simulink model "s_b4a4x32kf_54"  (R2018a)
(part 2 of 274)

  acc_len/1(in_reg) -> Delay21/1(d)
  [gbe_rxvld] -> pipeline76/1(d)
  [gbe_rxdata] -> pipeline75/1(d)
  [gbe_rxeof] -> pipeline77/1(d)
  gbe_porttx/1(in_reg) -> Delay9/1(d)
  gbe_iptx/1(in_reg) -> Delay10/1(d)
  Delay9/1(q) -> [gbe_porttx]
  Delay10/1(q) -> [gbe_iptx]
  board_id/1(in_reg) -> Delay72/1(d)
  unpack_feng_hardcoded/1(pkt_start) -> Terminator28/1
  unpack_feng_hardcoded/2(data256) -> pipeline34/1(d)
  unpack_feng_hardcoded/3(valid256) -> pipeline46/1(d)
  unpack_feng_hardcoded/4(eof256) -> pipeline47/1(d)
  Delay72/1(q) -> [board_id]
  vacc_time_msw/3(in_msw) -> Delay19/1(d)
  vacc_time_msw/1(in_arm) -> Delay16/1(d)
  Concat10/1 -> [vacc_ld_time]
  vacc_time_msw/2(in_immediate) -> Delay18/1(d)
  vacc_time_lsw/1(in_lsw) -> Delay20/1(d)
  Delay16/1(q) -> [vacc_ld_arm]
  Delay18/1(q) -> [vacc_ld_immediate]
  Delay19/1(q) -> Concat10/1
  Delay20/1(q) -> Concat10/2
  Delay21/1(q) -> [acc_len]
  pipeline24/1(q) -> [gap_size3]
  pipeline23/1(q) -> [gap_size2]
  pipeline14/1(q) -> [gap_size1]
  pipeline10/1(q) -> [gap_size0]
  gapsize/1(in_gap_size) -> Register/1, Relational/2, Delay1/1
  Delay1/1 -> Relational/1
  Register/1 -> pipeline24/1(d), pipeline23/1(d), pipeline14/1(d), pipeline10/1(d)
  bf_config/1(in_data_id) -> pipeline26/1(d)
  bf_config/2(in_time_id) -> pipeline27/1(d)
  bf_weight/1(in_stream) -> pipeline29/1(d)
  bf_weight/2(in_antenna) -> pipeline30/1(d)
  pipeline26/1(q) -> [bf_data_id]
  pipeline27/1(q) -> [bf_time_id]
  pipeline29/1(q) -> [bf_stream]
  pipeline30/1(q) -> [bf_antenna]
  pipeline55/1(q) -> [bf_value_bw]
  pipeline33/1(q) -> edge_detect7/1(in)
  [bfout_valbw0] -> Delay27/1(d)
  [bfout_valbw1] -> Delay26/1(d)
  [bfout_valbw2] -> Delay28/1(d)
  [bfout_valbw3] -> Delay32/1(d)
  Delay27/1(q) -> bf_valout_bw0/1(out_bw0)
  Delay26/1(q) -> bf_valout_bw0/2(out_bw1)
  Delay32/1(q) -> bf_valout_bw1/2(out_bw3)
  Delay28/1(q) -> bf_valout_bw1/1(out_bw2)
  edge_detect7/1(out) -> [bf_valctrl_bw]
  pipeline59/1(q) -> [bf_tvgsel]
  bf_config/3(in_tvg_sel) -> pipeline59/1(d)
  pipeline60/1(q) -> [bf_snap_arm]
  pipeline61/1(q) -> [bf_snap_trig]
  bf_config/4(in_snap_arm) -> pipeline60/1(d)
  bf_config/5(in_snap_trig) -> pipeline61/1(d)
  pipeline43/1(q) -> [bf1_txport]
  pipeline44/1(q) -> [bf1_txen]
  pipeline35/1(q) -> [bf0_txport]
  pipeline36/1(q) -> [bf0_txen]
  pipeline51/1(q) -> [bf0_txip]
  pipeline52/1(q) -> [bf1_txip]
  pipeline73/1(q) -> Convert/1
  pipeline74/1(q) -> Convert1/1
  gbe0/1(led_up) -> [gbe_up]
  gbe0/2(led_rx) -> Terminator1/1
  gbe0/3(led_tx) -> Terminator6/1
  gbe0/4(tx_afull) -> Terminator8/1
  gbe0/5(tx_overflow) -> [gbe_tx_over]
  gbe0/6(rx_data) -> [gbe_rxdata]
  gbe0/8(rx_source_ip) -> [gbe_src_ip]
  gbe0/9(rx_source_port) -> [gbe_src_port]
  gbe0/10(rx_end_of_frame) -> [gbe_rxeof]
  gbe0/11(rx_bad_frame) -> [gbe_rx_bad]
  gbe0/12(rx_overrun) -> [gbe_rx_overrun]
  gbe0/14(rx_dest_port) -> [gbe_dest_port]
  gbe0/13(rx_dest_ip) -> [gbe_dest_ip]
  [gbe_rst] -> gbe0/1(rst)
  [gbe_txd] -> gbe0/2(tx_data)
  [gbe_txip] -> gbe0/4(tx_dest_ip)
  [gbe_txport] -> gbe0/5(tx_dest_port)
  [gbe_txeof] -> gbe0/6(tx_end_of_frame)
  Constant3/1 -> gbe0/7(rx_ack)
  Constant4/1 -> gbe0/8(rx_overrun_ack)
  [gbe_debug_rst] -> gbe0/9(debug_rst)
  unpack_feng_hardcoded/13(hdr5_0x1600_DIR) -> pipeline49/1(d)
  unpack_feng_hardcoded/9(hdr_heap_id) -> Terminator2/1
  unpack_feng_hardcoded/10(hdr_heap_size) -> Terminator3/1
  unpack_feng_hardcoded/11(hdr_heap_offset) -> pipeline48/1(d)
  unpack_feng_hardcoded/12(hdr_pkt_len) -> Terminator5/1
  unpack_feng_hardcoded/14(hdr6_0x4101_DIR) -> pipeline53/1(d)
  unpack_feng_hardcoded/16(hdr8_0x4300) -> Terminator31/1
  unpack_feng_hardcoded/15(hdr7_0x4103_DIR) -> pipeline56/1(d)
  pipeline77/1(q) -> unpack_feng_hardcoded/3(pkt_eof)
  pipeline76/1(q) -> unpack_feng_hardcoded/2(pkt_valid)
  pipeline75/1(q) -> unpack_feng_hardcoded/1(pkt_data)
  Concat8/1 -> gbe_mux_bus/1(di)
  [pack_txd1] -> Concat8/2
  [pack_txd0] -> Concat8/1
  Concat11/1 -> gbe_mux_bus/2(validi)
  Concat2/1 -> gbe_mux_bus/3(eofi)
  gbe_mux_bus/5(start) -> bus_expand1/1(bus_in), Delay6/1
  Concat3/1 -> gbe_mux_bus/4(drdy)
  Constant2/1 -> gbe_mux_bus/5(transmit)
  gbe_mux_bus/2(do) -> Delay7/1
  gbe_mux_bus/3(valido) -> Delay17/1
  gbe_mux_bus/4(eofo) -> Delay25/1
  gbe_mux_bus/6(flush) -> [flush]
  [bf0s_d0] -> Concat8/3
  [bf1s_d0] -> Concat8/4
  [pack_txvld0] -> Concat11/1
  [pack_txvld1] -> Concat11/2
  [bf0s_en0] -> Concat11/3
  [bf1s_en0] -> Concat11/4
  [bf0s_eof0] -> Concat2/3
  [bf1s_eof0] -> Concat2/4
  [pack_txeof0] -> Concat2/1
  [pack_txeof1] -> Concat2/2
  [bf0s_pkt_ready0] -> Concat3/3
  [bf1s_pkt_ready0] -> Concat3/4
  [pack_ready1] -> Concat3/2
  [pack_ready0] -> Concat3/1
  [bf0s_d1] -> Concat8/5
  [bf1s_d1] -> Concat8/6
  [bf0s_en1] -> Concat11/5
  [bf1s_en1] -> Concat11/6
  [bf0s_eof1] -> Concat2/5
  [bf1s_eof1] -> Concat2/6
  [bf0s_pkt_ready1] -> Concat3/5
  [bf1s_pkt_ready1] -> Concat3/6
  Delay7/1 -> [gbe_txd]
  Delay17/1 -> [gbe_txvld]
  Delay25/1 -> [gbe_txeof]
  [bf0_txport] -> Mux6/6, Mux6/4
  [bf1_txport] -> Mux6/5, Mux6/7
  [gbe_porttx] -> Mux6/3, Mux6/2
  Mux6/1 -> [gbe_txport]
  gbe_mux_bus/1(input) -> [gbe_ipsel]
  Delay6/1 -> [gbe_txstart]
  Mux5/1 -> [gbe_txip]
  [bf0_txport] -> Mux6/12, Mux6/10
  [bf1_txport] -> Mux6/13, Mux6/11
  [gbe_porttx] -> Mux6/9, Mux6/8
  bus_expand1/12(lsb_out1) -> [bf1_tx_pkt3]
  bus_expand1/1(msb_out12) -> [go0]
  bus_expand1/2(out11) -> [go1]
  bus_expand1/3(out10) -> [bf0_tx_pkt0]
  bus_expand1/4(out9) -> [bf1_tx_pkt0]
  bus_expand1/5(out8) -> [bf0_tx_pkt1]
  bus_expand1/6(out7) -> [bf1_tx_pkt1]
  bus_expand1/7(out6) -> [go2]
  bus_expand1/8(out5) -> [go3]
  bus_expand1/9(out4) -> [bf0_tx_pkt2]
  bus_expand1/10(out3) -> [bf1_tx_pkt2]
  bus_expand1/11(out2) -> [bf0_tx_pkt3]
  [gbe_iptx] -> Concat/1
  [gbe_iptx] -> Concat/2
  [bf0_txip] -> Concat/3
  [bf1_txip] -> Concat/4
  [bf0_txip] -> Concat/5
  [bf1_txip] -> Concat/6
  [gbe_iptx] -> Concat/7
  [gbe_iptx] -> Concat/8
  [bf0_txip] -> Concat/9
  [bf1_txip] -> Concat/10
  [bf0_txip] -> Concat/11
  [bf1_txip] -> Concat/12
  Concat/1 -> bus_addsub/1(a)
  [id2] -> Concat1/9
  [id3] -> Concat1/12
  [id1] -> Concat1/2
  [id0] -> Concat1/1
  [id1] -> Concat1/5
  [id0] -> Concat1/4
  [id3] -> Concat1/8
  [id1] -> Concat1/6
  [id3] -> Concat1/11
  [id2] -> Concat1/10
  [id0] -> Concat1/3
  [id2] -> Concat1/7
  Concat1/1 -> bus_addsub/2(b)
  bus_addsub/1(dout) -> bus_expand/1(bus_in)
  bus_expand/1(msb_out12) -> Mux5/2
  bus_expand/2(out11) -> Mux5/3
  bus_expand/3(out10) -> Mux5/4
  bus_expand/4(out9) -> Mux5/5
  bus_expand/5(out8) -> Mux5/6
  bus_expand/6(out7) -> Mux5/7
  bus_expand/7(out6) -> Mux5/8
  bus_expand/8(out5) -> Mux5/9
  bus_expand/9(out4) -> Mux5/10
  bus_expand/10(out3) -> Mux5/11
  bus_expand/11(out2) -> Mux5/12
  bus_expand/12(lsb_out1) -> Mux5/13
  [pack_txd2] -> Concat8/7
  [pack_txd3] -> Concat8/8
  [pack_txvld2] -> Concat11/7
  [pack_txvld3] -> Concat11/8
  [pack_txeof2] -> Concat2/7
  [pack_txeof3] -> Concat2/8
  [pack_ready2] -> Concat3/7
  [pack_ready3] -> Concat3/8
  [bf0s_d2] -> Concat8/9
  [bf1s_d2] -> Concat8/10
  [bf0s_d3] -> Concat8/11
  [bf1s_d3] -> Concat8/12
  [bf0s_en2] -> Concat11/9
  [bf1s_en2] -> Concat11/10
  [bf0s_en3] -> Concat11/11
  [bf1s_en3] -> Concat11/12
  [bf0s_eof2] -> Concat2/9
  [bf1s_eof2] -> Concat2/10
  [bf0s_eof3] -> Concat2/11
  [bf1s_eof3] -> Concat2/12
  [bf0s_pkt_ready2] -> Concat3/9
  [bf1s_pkt_ready2] -> Concat3/10
  [bf0s_pkt_ready3] -> Concat3/11
  [bf1s_pkt_ready3] -> Concat3/12
  Relational/1 -> Register/2
  [gbe_ipsel] -> Mux5/1
  [gbe_ipsel] -> Mux6/1
  [gbe_txvld] -> gbe0/3(tx_valid)
  gbe0/7(rx_valid) -> [gbe_rxvld]
  unpack_feng_hardcoded/5(magic_error) -> [spead_magic_err]
  unpack_feng_hardcoded/6(hdr_error) -> [spead_hdr_err]
  unpack_feng_hardcoded/7(pad_error) -> [spead_pad_err]
  unpack_feng_hardcoded/8(pkt_len_err) -> [spead_pkt_len_err]
  [spead_pkt_len_err] -> Subsystem2/5(in3)
  [spead_pad_err] -> Subsystem2/4(in2)
  Subsystem2/4(out3) -> spead_status0/4(out_pkt_len_err_cnt)
  Subsystem2/3(out2) -> spead_status0/3(out_pad_err_cnt)
  Subsystem2/2(out1) -> spead_status0/2(out_header_err_cnt)
  Subsystem2/1(out0) -> spead_status0/1(out_magic_err_cnt)
  [cnt_rst] -> Subsystem2/1(rst)
  [spead_magic_err] -> Subsystem2/2(in0)
  [spead_hdr_err] -> Subsystem2/3(in1)
  [gbe_rxvld] -> Delay48/1
  [gbe_rxdata] -> Slice5/1
  [gbe_rxeof] -> Delay49/1
  [gbe_dest_ip] -> Delay50/1
  [gbe_rx_overrun] -> Delay55/1
  [gbe_src_ip] -> Delay52/1
  [gbe_dest_port] -> Delay51/1
  [gbe_src_port] -> Delay53/1
  [gbe_rx_bad] -> Delay54/1
  [gbe_rxvld] -> Delay56/1
  [gbe_rxeof] -> Delay57/1
  [spead_pkt_len_err] -> Logical4/4
  [spead_pad_err] -> Logical4/3
  [spead_hdr_err] -> Logical4/2
  [spead_magic_err] -> Logical4/1
  Logical4/1 -> snap_gbe0_rx/12(stop)
  Delay47/1 -> snap_gbe0_rx/1(in_data)
  Delay48/1 -> snap_gbe0_rx/2(in_valid)
  Delay49/1 -> snap_gbe0_rx/3(in_eof)
  Delay50/1 -> snap_gbe0_rx/4(in_dest_ip)
  Delay51/1 -> snap_gbe0_rx/5(in_dest_port)
  Delay52/1 -> snap_gbe0_rx/6(in_src_ip)
  Delay53/1 -> snap_gbe0_rx/7(in_src_port)
  Delay54/1 -> snap_gbe0_rx/8(in_rx_bad)
  Delay55/1 -> snap_gbe0_rx/9(in_rx_over)
  Delay56/1 -> snap_gbe0_rx/10(we)
  Delay57/1 -> snap_gbe0_rx/11(trig)
  Delay58/1 -> snap_gbe0_rx/13(arm)
  Slice5/1 -> Delay47/1
  [gbe_ipsel] -> Delay81/1
  [gbe_txeof] -> snap_pack_mux/2(in_eof)
  Delay81/1 -> snap_pack_mux/1(in_input_select)
  [gbe_txvld] -> snap_pack_mux/52(we)
  [go3] -> snap_pack_mux/6(in_go3)
  [go2] -> snap_pack_mux/5(in_go2)
  [go1] -> snap_pack_mux/4(in_go1)
  [go0] -> snap_pack_mux/3(in_go0)
  [bf0_tx_pkt0] -> snap_pack_mux/7(in_bf0_tx_pkt0)
  [bf0_tx_pkt1] -> snap_pack_mux/8(in_bf0_tx_pkt1)
  [bf0_tx_pkt2] -> snap_pack_mux/9(in_bf0_tx_pkt2)
  [bf0_tx_pkt3] -> snap_pack_mux/10(in_bf0_tx_pkt3)
  [bf1_tx_pkt0] -> snap_pack_mux/11(in_bf1_tx_pkt0)
  [bf1_tx_pkt1] -> snap_pack_mux/12(in_bf1_tx_pkt1)
  [bf1_tx_pkt2] -> snap_pack_mux/13(in_bf1_tx_pkt2)
  [bf1_tx_pkt3] -> snap_pack_mux/14(in_bf1_tx_pkt3)
  [pack_ready0] -> snap_pack_mux/15(in_rdy0)
  [pack_ready1] -> snap_pack_mux/16(in_rdy1)
  [pack_ready2] -> snap_pack_mux/17(in_rdy2)
  [pack_ready3] -> snap_pack_mux/18(in_rdy3)
  [bf0s_pkt_ready0] -> snap_pack_mux/19(in_bf0_rdy0)
  [bf0s_pkt_ready1] -> snap_pack_mux/20(in_bf0_rdy1)
  [bf0s_pkt_ready2] -> snap_pack_mux/21(in_bf0_rdy2)
  [bf0s_pkt_ready3] -> snap_pack_mux/22(in_bf0_rdy3)
  [bf1s_pkt_ready0] -> snap_pack_mux/23(in_bf1_rdy0)
  [bf1s_pkt_ready1] -> snap_pack_mux/24(in_bf1_rdy1)
  [bf1s_pkt_ready2] -> snap_pack_mux/25(in_bf1_rdy2)
  [bf1s_pkt_ready3] -> snap_pack_mux/26(in_bf1_rdy3)
  [bf1s_en0] -> snap_pack_mux/35(in_bf1_vld0)
  [pack_txvld3] -> snap_pack_mux/30(in_vld3)
  [pack_txvld0] -> snap_pack_mux/27(in_vld0)
  [bf1s_en3] -> snap_pack_mux/38(in_bf1_vld3)
  [bf0s_en1] -> snap_pack_mux/32(in_bf0_vld1)
  [pack_txvld1] -> snap_pack_mux/28(in_vld1)
  [bf0s_en0] -> snap_pack_mux/31(in_bf0_vld0)
  [bf0s_en3] -> snap_pack_mux/34(in_bf0_vld3)
  [pack_txvld2] -> snap_pack_mux/29(in_vld2)
  [bf0s_en2] -> snap_pack_mux/33(in_bf0_vld2)
  [bf1s_en2] -> snap_pack_mux/37(in_bf1_vld2)
  [bf1s_en1] -> snap_pack_mux/36(in_bf1_vld1)
  [bf1s_eof3] -> snap_pack_mux/50(in_bf1_eof3)
  [bf0s_eof2] -> snap_pack_mux/45(in_bf0_eof2)
  [bf0s_eof0] -> snap_pack_mux/43(in_bf0_eof0)
  [pack_txeof3] -> snap_pack_mux/42(in_eof3)
  [bf1s_eof1] -> snap_pack_mux/48(in_bf1_eof1)
  [pack_txeof0] -> snap_pack_mux/39(in_eof0)
  [bf0s_eof1] -> snap_pack_mux/44(in_bf0_eof1)
  [pack_txeof2] -> snap_pack_mux/41(in_eof2)
  [bf0s_eof3] -> snap_pack_mux/46(in_bf0_eof3)
  [bf1s_eof2] -> snap_pack_mux/49(in_bf1_eof2)
  [bf1s_eof0] -> snap_pack_mux/47(in_bf1_eof0)
  [pack_txeof1] -> snap_pack_mux/40(in_eof1)
  [gbe_txeof] -> snap_pack_mux/53(trig)
  [gbe_txip] -> Slice/1
  Slice/1 -> snap_pack_mux/51(in_ip)
  pipeline65/1(q) -> [vacctvg_sync_sel]
  pipeline62/1(q) -> [vacctvg_valid_sel]
  pipeline64/1(q) -> [vacctvg_reset]
  pipeline66/1(q) -> [vacctvg_data_sel]
  pipeline67/1(q) -> [vacctvg_vector_en]
  pipeline69/1(q) -> [vacctvg_ctr_en]
  pipeline70/1(q) -> [vacctvg_pulse_en]
  pipeline68/1(q) -> [vacctvg_run]
  tvg_control/12(in_reord_snap_dv_mux) -> pipeline7/1(d)
  tvg_control/14(in_reord_snap_dv_arm) -> pipeline11/1(d)
  tvg_control/15(in_preproc_snap_dv_mux) -> pipeline15/1(d)
  pipeline7/1(q) -> [reord_snap_dv_mux]
  pipeline11/1(q) -> [reord_snap_dv_arm]
  pipeline15/1(q) -> [preproc_snap_dv_mux]
  pipeline16/1(q) -> [snap_hmc_reord_stop_sel]
  pipeline9/1(q) -> [xeng_tvg_data_sel]
  tvg_control/13(in_xeng_tvg_data_sel) -> pipeline9/1(d)
  tvg_control/17(in_xeng_tvg_val_sel) -> pipeline17/1(d)
  tvg_control/18(in_xeng_tvg_inj_vector) -> pipeline18/1(d)
  tvg_control/19(in_xeng_tvg_mcnt_sel) -> pipeline19/1(d)
  pipeline17/1(q) -> [xeng_tvg_val_sel]
  pipeline18/1(q) -> [xengtvg_inj_vector]
  pipeline19/1(q) -> [xeng_tvg_mcnt_sel]
  tvg_control/3(in_vacc_tvg_sync_sel) -> pipeline65/1(d)
  tvg_control/4(in_vacc_tvg_valid_sel) -> pipeline62/1(d)
  tvg_control/5(in_vacc_tvg_data_sel) -> pipeline66/1(d)
  tvg_control/6(in_vacc_tvg_reset) -> pipeline64/1(d)
  tvg_control/7(in_vacc_tvg_ctr_en) -> pipeline69/1(d)
  tvg_control/10(in_vacc_tvg_vector_en) -> pipeline67/1(d)
  tvg_control/11(in_vacc_tvg_run) -> pipeline68/1(d)
  tvg_control/2(in_vacc_tvg_pulse_en) -> pipeline70/1(d)
  tvg_control/20(in_preproc_snap_stop_mux) -> pipeline20/1(d)
  pipeline20/1(q) -> [preproc_snap_stop_mux]
  pipeline37/1(q) -> [snp_hmc_pkt_mux_we_sel]
  pipeline39/1(q) -> [snp_reord_mux_we_sel]
  tvg_control/22(in_snap_reord_mux_we_sel) -> pipeline39/1(d)
  tvg_control/21(in_snap_hmc_pkt_reord_we_sel) -> pipeline37/1(d)
  [hmc_reord_data] -> Slice1/1
  [hmc_reord_valid] -> Delay4/1
  [hmc_reord_timestamp] -> Slice6/1
  Slice1/1 -> Delay3/1
  Slice6/1 -> Delay8/1
  [hmc_reord_fengid] -> Delay30/1
  [hmc_reord_freq] -> Delay31/1
  [hmc_reord_pkt_idx] -> Delay5/1
  [hmc_pkt_reord_err] -> Delay35/1
  Delay3/1 -> snap_hmc_pkt_reord/1(in_data)
  Delay4/1 -> snap_hmc_pkt_reord/2(in_valid)
  Delay8/1 -> snap_hmc_pkt_reord/4(in_timestamp)
  Delay30/1 -> snap_hmc_pkt_reord/5(in_fengid)
  Delay43/1 -> snap_hmc_pkt_reord/9(we)
  Delay37/1 -> snap_hmc_pkt_reord/11(stop)
  Delay36/1 -> snap_hmc_pkt_reord/10(trig)
  Delay5/1 -> snap_hmc_pkt_reord/3(in_pkt_idx)
  Delay31/1 -> snap_hmc_pkt_reord/6(in_freq)
  Delay33/1 -> snap_hmc_pkt_reord/7(in_xeng)
  Delay35/1 -> snap_hmc_pkt_reord/8(in_err)
  [hmc_reord_xeng] -> Delay33/1
  [hmc_pkt_reord_rd_start_g] -> Delay36/1
  [hmc_pkt_reord_err] -> Delay37/1
  [hmc_reord_xeng] -> Relational1/1
  Constant/1 -> Relational1/2
  [snp_hmc_pkt_mux_we_sel] -> Delay38/1
  [hmc_reord_valid] -> Delay40/1
  Logical3/1 -> Mux/3
  Relational1/1 -> Logical8/2, Logical3/1
  Delay38/1 -> Delay41/1
  Delay41/1 -> Mux/1
  Delay42/1 -> Mux/2
  Mux/1 -> Delay43/1
  [spead_pkt_len_err] -> Logical2/4
  [spead_pad_err] -> Logical2/3
  [spead_hdr_err] -> Logical2/2
  [spead_magic_err] -> Logical2/1
  Slice2/1 -> Delay/1
  Slice3/1 -> Delay12/1
  Slice4/1 -> Delay13/1
  Logical2/1 -> Delay59/1, Delay34/1
  pipeline46/1(q) -> [spead_valid]
  pipeline47/1(q) -> [spead_eof]
  Delay/1 -> snap_rx_unpack0/1(in_data)
  Delay2/1 -> snap_rx_unpack0/2(in_valid), Logical5/1
  Delay12/1 -> Register1/1, snap_rx_unpack0/4(in_timestamp)
  Delay13/1 -> snap_rx_unpack0/5(in_fengid)
  Delay11/1 -> snap_rx_unpack0/3(in_eof), Logical5/2
  Delay34/1 -> snap_rx_unpack0/10(stop)
  Delay39/1 -> snap_rx_unpack0/9(trig)
  Delay14/1 -> snap_rx_unpack0/7(in_xeng_id)
  Delay44/1 -> snap_rx_unpack0/6(in_freq_this_eng)
  freq_this_eng_in/1 -> Delay44/1
  xeng_id/1 -> Delay14/1
  Delay59/1 -> [unpack_err_g]
  Logical5/1 -> snap_rx_unpack0/8(we)
  Logical8/1 -> Mux/4
  Delay29/1 -> Relational2/2
  Relational2/1 -> Logical8/3
  [hmc_reord_timestamp] -> Relational2/1, Delay29/1
  Relational3/1 -> Logical9/3
  Constant20/1 -> Relational3/2
  [hmc_reord_pkt_idx] -> Relational3/1
  Delay40/1 -> Logical9/1, Logical8/1, Logical3/2, Delay42/1
  Logical9/1 -> Mux/5
  [hmc_pkt_reord_err] -> Delay15/1
  Delay15/1 -> Logical9/2
  snap_rx_unpack0/1(arm_out) -> edge_detect8/1(in), Delay58/1, snap_hmc_pkt_reord/12(arm)
  edge_detect8/1(out) -> Register1/2
  Register1/1 -> Relational4/2
  [hmc_reord_timestamp] -> Relational4/1
  Relational4/1 -> Logical12/1
  [hmc_pkt_reord_err] -> Logical12/2
  Logical12/1 -> Logical2/5
  spead_time_check/1(err_cnt) -> spead_status0/5(out_time_err_cnt)
  Subsystem11/1(out0) -> spead_status1/1(out_valid_pkt_cnt)
  pipeline49/1(q) -> [spead_timestamp]
  [spead_timestamp] -> spead_time_check/2(timestamp)
  [spead_valid] -> spead_time_check/3(valid)
  [spead_valid] -> Subsystem11/3(valid)
  [spead_eof] -> Subsystem11/2(eof)
  [cnt_rst] -> Subsystem11/1(rst)
  [cnt_rst] -> spead_time_check/1(cnt_rst)
  [spead_timestamp] -> Slice3/1
  [spead_valid] -> Delay2/1
  [spead_eof] -> Delay11/1
  [spead_eof] -> Delay39/1
  pipeline48/1(q) -> [spead_heap_offset]
  [spead_heap_offset] -> freq_this_eng_in/1
  pipeline53/1(q) -> [spead_feng_id]
  [spead_feng_id] -> Slice4/1
  pipeline56/1(q) -> [spead_freq_base]
  pipeline34/1(q) -> [spead_data]
  [spead_data] -> Slice2/1
  [spead_freq_base] -> xeng_id/1
  pipeline21/1(q) -> [snap_reord_mux_stop_sel]
  tvg_control/23(in_snap_reord_mux_stop_sel) -> pipeline21/1(d)
  tvg_control/16(in_snap_hmc_reord_stop_sel) -> pipeline16/1(d)
  bf_weight/3(in_load_now) -> pipeline33/1(d)
  bf_weight/4(in_weight) -> pipeline55/1(d)
  bf1_ip/1(in_ip) -> pipeline52/1(d)
  bf0_ip/1(in_ip) -> pipeline51/1(d)
  bf0_config/1(in_quant_gain) -> pipeline73/1(d)
  bf0_config/2(in_port) -> pipeline35/1(d)
  bf0_config/3(in_txen) -> pipeline36/1(d)
  bf1_config/3(in_txen) -> pipeline44/1(d)
  bf1_config/2(in_port) -> pipeline43/1(d)
  bf1_config/1(in_quant_gain) -> pipeline74/1(d)
  Convert/1 -> [bf0_gain]
  Convert1/1 -> [bf1_gain]
  xeng_tx_offset0/1(in_tx_offset) -> Delay22/1
  Delay22/1 -> [xeng_tx_offset0]
  Delay23/1 -> [xeng_tx_offset1]
  xeng_tx_offset1/1(in_tx_offset) -> Delay23/1
  Delay24/1 -> [xeng_tx_offset2]
  xeng_tx_offset2/1(in_tx_offset) -> Delay24/1
  Delay45/1 -> [xeng_tx_offset3]
  xeng_tx_offset3/1(in_tx_offset) -> Delay45/1
  tvg_control/8(in_vacc_tvg_ctr2_en) -> pipeline22/1(d)
  pipeline22/1(q) -> [vacctvg_ctr2_en]
  tvg_control/1(in_vacc_tvg_time_sel) -> pipeline28/1(d)
  pipeline28/1(q) -> [vacctvg_time_sel]
  tvg_control/9(in_vacc_tvg_ctr3_en) -> pipeline31/1(d)
  pipeline31/1(q) -> [vacctvg_ctr3_en]
  pipeline2/1(q) -> [gbe_rst]
  pipeline8/1(q) -> [flasher_en]
  control/6(in_flasher_en) -> pipeline8/1(d)
  pipeline12/1(q) -> [auto_rst_en]
  edge_detect5/1(out) -> [reord_snaptrig]
  control/9(in_unpack_snapwesel) -> pipeline25/1(d)
  pipeline4/1(q) -> edge_detect1/1(in)
  pipeline13/1(q) -> [reord_snaptrigsel]
  control/7(in_reord_snaptrig) -> pipeline6/1(d)
  edge_detect1/1(out) -> [gbe_debug_rst]
  control/3(in_gbe_rst) -> pipeline2/1(d)
  pipeline25/1(q) -> [unpack_snapwesel]
  control/5(in_gbe_debug_rst) -> pipeline4/1(d)
  edge_detect/1(out) -> [cnt_rst]
  control/8(in_reord_snaptrigsel) -> pipeline13/1(d)
  control/4(in_gbe_txen) -> pipeline5/1(d)
  control/1(in_auto_rst_enable) -> pipeline12/1(d)
  pipeline5/1(q) -> [gbe_txen]
  control/2(in_cnt_rst) -> pipeline3/1(d)
  pipeline3/1(q) -> edge_detect/1(in)
  pipeline6/1(q) -> edge_detect5/1(in)
  Logical1/1 -> Subsystem7/1(dv)
  [spead_eof] -> Logical1/1
  Subsystem7/1(per_sec) -> spead_status2/1(out_pkts_per_sec)
  [spead_valid] -> Logical1/2
  [hmc_reord_valid] -> missing_ant_acc/4(valid)
  missing_ant_acc/3(we) -> missing_ant_cnts/3(we)
  hmc_pkt_reord/6(dest_xeng_this_brd) -> [hmc_reord_xeng]
  missing_ant_acc/2(data) -> missing_ant_cnts/2(data_in)
  hmc_pkt_reord/7(pkt_idx) -> [hmc_reord_pkt_idx]
  hmc_pkt_reord/5(freq_this_eng) -> [hmc_reord_freq]
  [spead_heap_offset] -> hmc_pkt_reord/6(heap_offset)
  hmc_pkt_reord/8(err) -> [hmc_pkt_reord_err]
  missing_ant_cnts/1(data_out) -> missing_ant_acc/5(In2)
  [hmc_reord_fengid] -> missing_ant_acc/1(ant)
  hmc_pkt_reord/3(timestamp) -> [hmc_reord_timestamp]
  [board_id] -> hmc_pkt_reord/8(board_id)
  [spead_timestamp] -> hmc_pkt_reord/4(spead_time48)
  missing_ant_acc/1(addr) -> missing_ant_cnts/1(addr)
  [hmc_reord_pkt_idx] -> missing_ant_acc/3(pkt_idx)
  [spead_data] -> hmc_pkt_reord/1(data_in)
  hmc_pkt_reord/1(data_out) -> [hmc_reord_data]
  hmc_pkt_reord/2(valid) -> [hmc_reord_valid]
  [spead_freq_base] -> hmc_pkt_reord/7(freq_base)
  hmc_pkt_reord/4(src_feng) -> [hmc_reord_fengid]
  [hmc_pkt_reord_missing] -> missing_ant_acc/2(err)
  [spead_feng_id] -> hmc_pkt_reord/5(spead_fengid)
  [spead_valid] -> hmc_pkt_reord/2(valid_in)
  hmc_pkt_reord/9(missing) -> [hmc_pkt_reord_missing]
  [spead_eof] -> hmc_pkt_reord/3(eof_in)
